simulink model "acc_ctrl_ref"  (R2024b)
settings: Solver=FixedStepDiscrete  StartTime=0.0  StopTime=T_sim  FixedStep=Ts  RelTol=1e-3
values from neighbouring files (symbols this model uses):
  Ts = 0.01    [acc_params.m]    (also in build_acc_controller.m = %g;', v_set, a_max, a_min, Ts); build_acc_plant.m)
settings Model: Creator=Aymen  LastModifiedBy=Aymen
settings DataIOCC: SaveOutput=off  SaveTime=off
settings OptimizationCC: DefaultParameterBehavior=Inlined  EnhancedBackFolding=on  PassReuseOutputArgsAs=Individual arguments  ZeroExternalMemoryAtStartup=off  ZeroInternalMemoryAtStartup=off  OptimizeBlockOrder=speed  DifferentSizesBufferReuse=on  OptimizationCustomize=off  EfficientTunableParamExpr=on
settings DebuggingCC: ParameterTunabilityLossMsg=error
settings SFSimCC: MATLABDynamicMemAlloc=off
settings RTWCC: Description=Embedded Coder  SystemTargetFile=ert.tlc  TemplateMakefile=ert_default_tmf  GenerateReport=on
settings CodeAppCC: ForceParamTrailComments=on  IgnoreCustomStorageClasses=off  OperatorAnnotations=on  SimulinkDataObjDesc=on  SFDataObjDesc=on  InsertBlockDesc=on
settings ERTTargetCC: TargetLangStandard=C99 (ISO)  GenerateSampleERTMain=on  ERTCustomFileTemplate=example_file_process.tlc

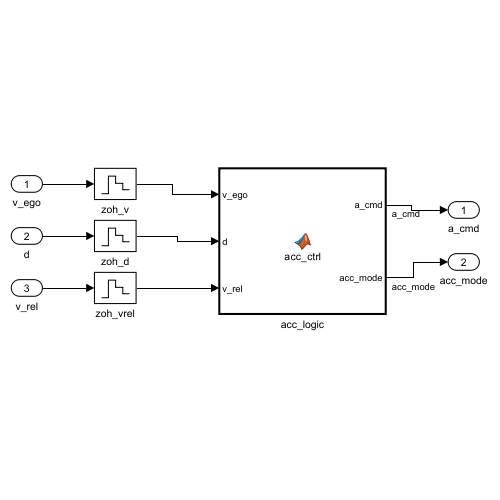
[thumbnail: Simulink's stored preview of the top-level diagram]
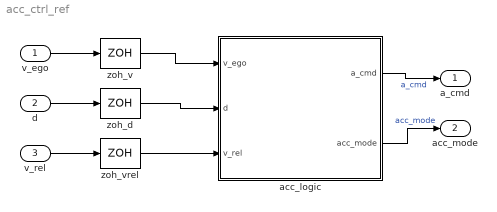
== system acc_ctrl_ref ==
  v_ego : Inport  OutDataTypeStr=double  PortDimensions=1  SampleTime=Ts
  d : Inport  Port=2  OutDataTypeStr=double  PortDimensions=1  SampleTime=Ts
  v_rel : Inport  Port=3  OutDataTypeStr=double  PortDimensions=1  SampleTime=Ts
  acc_logic : MATLAB Function  TreatAsAtomicUnit=on
  zoh_d : ZeroOrderHold  SampleTime=Ts
  zoh_v : ZeroOrderHold  SampleTime=Ts
  zoh_vrel : ZeroOrderHold  SampleTime=Ts
  a_cmd : Outport  OutDataTypeStr=double  PortDimensions=1  SampleTime=[0.01,0]
  acc_mode : Outport  Port=2  OutDataTypeStr=double  PortDimensions=1  SampleTime=[0.01,0]
  wires:
  v_ego/1 -> zoh_v/1
  d/1 -> zoh_d/1
  v_rel/1 -> zoh_vrel/1
  zoh_v/1 -> acc_logic/1(v_ego)
  zoh_d/1 -> acc_logic/2(d)
  zoh_vrel/1 -> acc_logic/3(v_rel)
  acc_logic/1(a_cmd) -> a_cmd/1  "a_cmd"
  acc_logic/2(acc_mode) -> acc_mode/1  "acc_mode"

== matlab function acc_ctrl_ref/acc_logic ==
  data: v_ego input; a_cmd output; d input; v_rel input; acc_mode output
function [a_cmd, acc_mode] = acc_ctrl(v_ego, d, v_rel)
% ACC : regulation de vitesse (PI) + suivi de distance (PD), selection par minimum
persistent integ
if isempty(integ)
    integ = 0;
end

% --- parametres (valeurs inscrites a la construction du modele) ---
v_set = 30;  a_max = 3;  a_min = -3;  Ts = 0.01;
Kp_v = 0.5;  Ki_v = 0.1;
th = 1.8;  d0 = 5;  d_detect = 150;
Kd_gap = 0.25;  Kv_rel = 0.8;

% --- regulation de vitesse : PI ---
e_v      = v_set - v_ego;
a_cruise = Kp_v*e_v + integ;

% --- suivi de distance : ecart a la distance desiree + vitesse relative ---
d_des    = d0 + th*max(v_ego, 0);
a_follow = Kd_gap*(d - d_des) + Kv_rel*v_rel;
target   = d < d_detect;

% --- selection du mode : on retient la consigne la plus prudente ---
if target && (a_follow < a_cruise)
    acc_mode = 2;
    a_raw    = a_follow;
else
    acc_mode = 1;
    a_raw    = a_cruise;
end

% --- saturation de la demande d acceleration ---
a_cmd = min(max(a_raw, a_min), a_max);

% --- anti-windup : integration conditionnelle, gelee en mode suivi ---
sat_hi = a_raw > a_max;
sat_lo = a_raw < a_min;
if acc_mode == 1 && ~((sat_hi && e_v > 0) || (sat_lo && e_v < 0))
    integ = min(max(integ + Ki_v*e_v*Ts, a_min), a_max);
end
